simulink model "control_system"  (R2023b)
settings: Solver=VariableStepAuto  StartTime=0.0  StopTime=10.0  MaxStep=0.01  RelTol=1e-3
undefined symbols (not defined in the file): I
libraries: slpidlib x2, simulink_extras x1
settings Model: Creator=maxaz  LastModifiedBy=maxaz

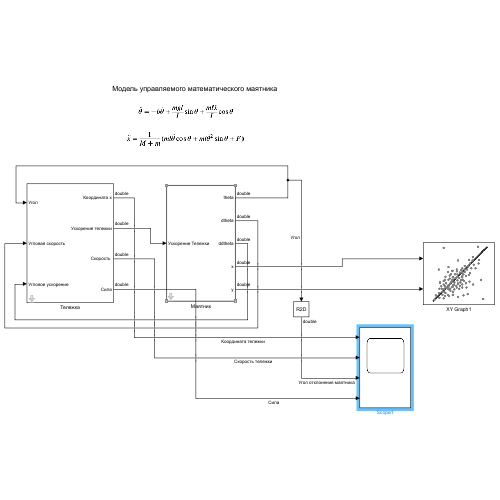
[thumbnail: Simulink's stored preview of the top-level diagram]
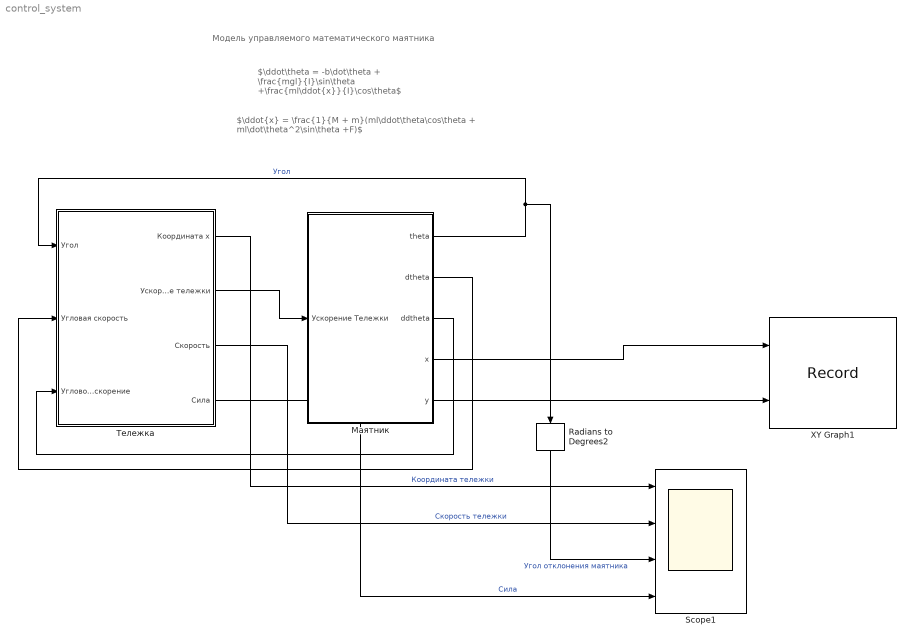
== system control_system ==
  note: Модель управляемого математического маятника
  note: $\ddot{x} = \frac{1}{M + m}(ml\ddot\theta\cos\theta + ml\dot\theta^2\sin\theta +F)$
  note: $\ddot\theta = -b\dot\theta + \frac{mgl}{I}\sin\theta +\frac{ml\ddot{x}}{I}\cos\theta$
  Radians to Degrees2 : simulink_extras/Transformations/Radians to Degrees
  Scope1 : Scope  NumInputPorts=4
  XY Graph1 : Record  FileSettingsInternal="{\"entries\":[{\"content\":{\"excelSettings\":{\"content\":{},\"type\":\"Streamout.ExcelSettings\"}},\"type\":\"Streamout.FileSettingStorage\",\"uuid\":\"\"}],\"packageUris\":[\"http:\\/\\/schema.mathworks.com\\/mf0\\/streamout_blocks\\/R2020a\"],\"version\":\"1.0\"}"  Layout=[1 1]  SignalsInternal="{\"entries\":[{\"content\":{\"signals\":[{\"content\":{\"blockPath\":[],\"dimensions\":[1],\"domain\":\"\",\"lineColor\":\"#a2142f\",\"plots\":[1],\"port\":1,\"sid\":[\"\"],\"signalID\":6168,\"signalName\":\"Маятник:4\"},\"type\":\"RecordBlkView.Signal\",\"uuid\":\"\"},{\"content\":{\"blockPath\":[],\"dimensions\":[1],\"domain\":\"\",\"lineColor\":\"#139fff\",\"plots\":[1],\"port\":2,\"sid\":[\"\"],\"signalID\":6172,\"signalName\":\"Маятник:5\"},\"type\":\"RecordBlkView.Signal\",\"uuid\":\"\"}]},\"type\":\"RecordBlkView.InputSignals\",\"uuid\":\"\"}],\"packageUris\":[\"http:\\/\\/schema.mathworks.com\\/mf0\\/streamout_blocks\\/R2020a\"],\"version\":\"1.0\"}"  VisualizationBindings="{\"xyplotplugin\":{\"info\":[{\"series\":[{\"bindingParametersList\":[{\"parameter\":\"X-Axis\",\"signalID\":6168,\"signalName\":\"Маятник:4\"},{\"parameter\":\"Y-Axis\",\"signalID\":6172,\"signalName\":\"Маятник:5\"}],\"seriesID\":9989}],\"subplotID\":1}]}}"  CompatibilityTag=XY
  Маятник : Subsystem  mask{m=1, g=9.8, l=1, startDegree=30, b=0.3}
      mask prompts: m "Масса, кг"; g "Ускорение свободного падения, м/с^2"; l "Длина, м"; startDegree "Начальный угол, градусы"; b "Диссипативный коэффициент"
  Тележка : Subsystem  mask{m=1, M_T=10, l=1, P=11, I=0, D=5.5}
      mask prompts: m "Масса маятника"; M_T "Масса тележки"; l "Длина маятника"
  wires:
  Тележка/4(Сила) -> Scope1/4  "Сила"
  Radians to Degrees2/1 -> Scope1/3  "Угол отклонения маятника"
  Тележка/3("Скорость ") -> Scope1/2  "Скорость тележки"
  Тележка/2(Ускорение тележки) -> Маятник/1(Ускорение Тележки)
  Маятник/3(ddtheta) -> Тележка/3(Угловое ускорение)
  Тележка/1(Координата x) -> Scope1/1  "Координата тележки"
  Маятник/2(dtheta) -> Тележка/2(Угловая скорость)
  Маятник/4(x) -> XY Graph1/1
  Маятник/5(y) -> XY Graph1/2
  Маятник/1(theta) -> Тележка/1(Угол), Radians to Degrees2/1  "Угол"

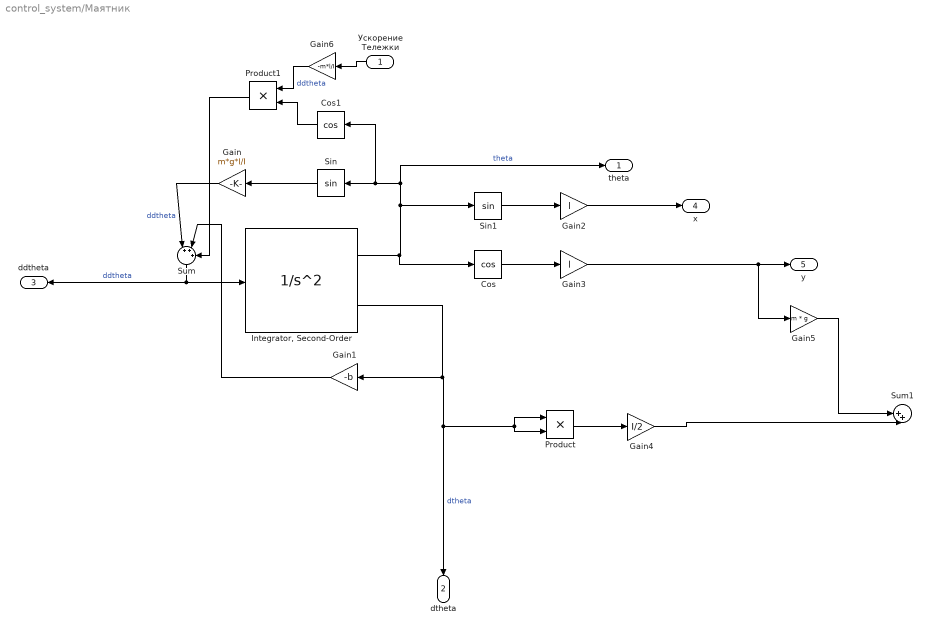
== system control_system/Маятник ==
  Ускорение Тележки : Inport
  Cos : Trigonometry  Operator=cos
  Cos1 : Trigonometry  Operator=cos
  Gain : Gain  Gain=m*g*l/I
  Gain1 : Gain  Gain=-b
  Gain2 : Gain  Gain=l
  Gain3 : Gain  Gain=l
  Gain4 : Gain  Gain=I/2
  Gain5 : Gain  Gain=m * g
  Gain6 : Gain  Gain=-m*l/I
  "Integrator, Second-Order" : SecondOrderIntegrator  ICX=deg2rad(startDegree)
  Product : Product
  Product1 : Product
  Sin : Trigonometry
  Sin1 : Trigonometry
  Sum : Sum  Inputs=|+++
  Sum1 : Sum  Inputs=|++
  theta : Outport
  dtheta : Outport  Port=2
  ddtheta : Outport  Port=3
  x : Outport  Port=4
  y : Outport  Port=5
  wires:
  "Integrator, Second-Order"/1 -> Cos/1, theta/1, Cos1/1, Sin/1, Sin1/1  "theta"
  Sin/1 -> Gain/1
  Sum/1 -> "Integrator, Second-Order"/1, ddtheta/1  "ddtheta"
  "Integrator, Second-Order"/2 -> Product/2, Product/1, dtheta/1, Gain1/1  "dtheta"
  Gain1/1 -> Sum/2
  Gain/1 -> Sum/1  "ddtheta"
  Cos/1 -> Gain3/1
  Gain2/1 -> x/1
  Sin1/1 -> Gain2/1
  Product/1 -> Gain4/1
  Gain5/1 -> Sum1/1
  Gain4/1 -> Sum1/2
  Gain3/1 -> Gain5/1, y/1
  Ускорение Тележки/1 -> Gain6/1
  Cos1/1 -> Product1/2
  Gain6/1 -> Product1/1  "ddtheta"
  Product1/1 -> Sum/3

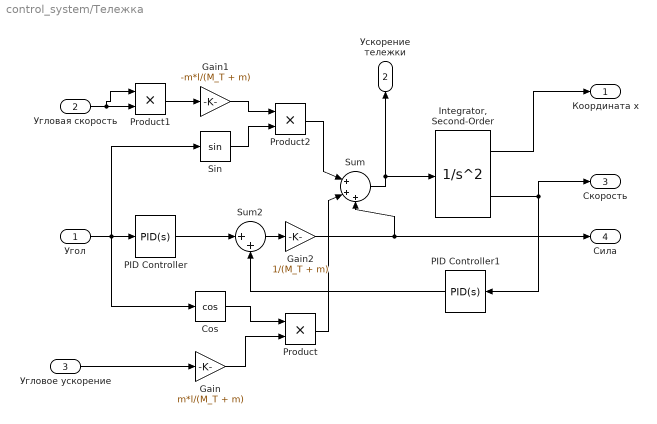
== system control_system/Тележка ==
  Угол : Inport
  Угловая скорость : Inport  Port=2
  Угловое ускорение : Inport  Port=3
  Cos : Trigonometry  Operator=cos
  Gain : Gain  Gain=m*l/(M_T + m)
  Gain1 : Gain  Gain=-m*l/(M_T + m)
  Gain2 : Gain  Gain=1/(M_T + m)
  "Integrator, Second-Order" : SecondOrderIntegrator
  PID Controller : slpidlib/PID Controller  Controller=PID  Form=Parallel  TimeDomain=Continuous-time  UseExternalTs=off  SampleTime=-1  IntegratorMethod=Forward Euler  FilterMethod=Forward Euler  ControllerParametersSource=internal  P=200  I=0  UseKiTs=off  D=50  N=100  UseFilter=on  TunerSelectOption=Transfer Function Based (PID Tuner App)  InitialConditionSource=internal  InitialConditionForIntegrator=0  InitialConditionForFilter=0  DifferentiatorICPrevScaledInput=0  ExternalReset=none  TrackingMode=off  Kt=1  LimitOutput=off  SatLimitsSource=internal  UpperSaturationLimit=inf  LowerSaturationLimit=-inf  LinearizeAsGain=on  AntiWindupMode=none  Kb=1  LimitIntegrator=off  UpperIntegratorSaturationLimit=inf  LowerIntegratorSaturationLimit=-inf  POutMin=[]  POutMax=[]  IOutMin=[]  IOutMax=[]  DOutMin=[]  DOutMax=[]  NOutMin=[]  NOutMax=[]  SumOutMin=[]  SumOutMax=[]  SaturationOutMin=[]  SaturationOutMax=[]  PParamMin=[]  PParamMax=[]  IParamMin=[]  IParamMax=[]  DParamMin=[]  DParamMax=[]  NParamMin=[]  NParamMax=[]  KbParamMin=[]  KbParamMax=[]  KtParamMin=[]  KtParamMax=[]  KbOutMin=[]  KbOutMax=[]  KtOutMin=[]  KtOutMax=[]  IntegratorOutMin=[]  IntegratorOutMax=[]  FilterOutMin=[]  FilterOutMax=[]  SumI1OutMin=[]  SumI1OutMax=[]  SumI2OutMin=[]  SumI2OutMax=[]  SumI3OutMin=[]  SumI3OutMax=[]  SumI4OutMin=[]  SumI4OutMax=[]  SumDOutMin=[]  SumDOutMax=[]  DifferentiatorOutMin=[]  DifferentiatorOutMax=[]  FilterDiffOutCoefMin=[]  FilterDiffOutCoefMax=[]  ReciprocalOutMin=[]  ReciprocalOutMax=[]  SumDenOutMin=[]  SumDenOutMax=[]  SumNumOutMin=[]  SumNumOutMax=[]  DivideOutMin=[]  DivideOutMax=[]  UdiffTsProdOutMin=[]  UdiffTsProdOutMax=[]  NTsProdOutMin=[]  NTsProdOutMax=[]  UintegralTsProdOutMin=[]  UintegralTsProdOutMax=[]  UngainTsProdOutMin=[]  UngainTsProdOutMax=[]  ClampingZeroOutDataTypeStr=Inherit: Inherit via back propagation  ClampingZeroOutMin=[]  ClampingZeroOutMax=[]  FilterDenConstantOutDataTypeStr=Inherit: Inherit via back propagation  FilterDenConstantOutMin=[]  FilterDenConstantOutMax=[]  PCopyOutDataTypeStr=Inherit: Inherit via back propagation  PCopyOutMin=[]  PCopyOutMax=[]  NCopyOutDataTypeStr=Inherit: Inherit via back propagation  NCopyOutMin=[]  NCopyOutMax=[]  IntegratorContinuousStateAttributes=''  IntegratorStateMustResolveToSignalObject=off  IntegratorRTWStateStorageClass=Auto  FilterContinuousStateAttributes=''  FilterStateMustResolveToSignalObject=off  FilterRTWStateStorageClass=Auto  ParallelPVariant=InternalParameters  IdealPVariant=Disabled  IVariant=InternalParameters  DVariant=InternalParameters  IntegratorVariant=Continuous  SatVariant=Disabled  AWVariant=Passthrough  PCopyVariant=Disabled  TRVariant=Disabled  FdbkBlocksVariant=Forward  IdealPFdbkVariant=Disabled  SatFdbkVariant=Disabled  DerivativeFilterVariant=ContFilter  NVariant=InternalParameters  NCopyVariant=Disabled  FilterICVariant=InternalICsFilter  IntegratorICVariant=InternalICs  ExternalResetVariant=Disabled  TRSumVariant=Passthrough  SumFdbkVariant=Disabled  SumVariant=Sum_PID  TsampFilterVariant=InternalTs  TsampNgainVariant=Passthrough  TsampIntegralVariant=Disabled_SignalSpec  ExternalSaturationOutDataTypeStr=Inherit: Same as second input
  PID Controller1 : slpidlib/PID Controller  Controller=PID  Form=Parallel  TimeDomain=Continuous-time  UseExternalTs=off  SampleTime=-1  IntegratorMethod=Forward Euler  FilterMethod=Forward Euler  ControllerParametersSource=internal  P=P  I=I  UseKiTs=off  D=D  N=100  UseFilter=on  TunerSelectOption=Transfer Function Based (PID Tuner App)  InitialConditionSource=internal  InitialConditionForIntegrator=0  InitialConditionForFilter=0  DifferentiatorICPrevScaledInput=0  ExternalReset=none  TrackingMode=off  Kt=1  LimitOutput=off  SatLimitsSource=internal  UpperSaturationLimit=inf  LowerSaturationLimit=-inf  LinearizeAsGain=on  AntiWindupMode=none  Kb=1  LimitIntegrator=off  UpperIntegratorSaturationLimit=inf  LowerIntegratorSaturationLimit=-inf  POutMin=[]  POutMax=[]  IOutMin=[]  IOutMax=[]  DOutMin=[]  DOutMax=[]  NOutMin=[]  NOutMax=[]  SumOutMin=[]  SumOutMax=[]  SaturationOutMin=[]  SaturationOutMax=[]  PParamMin=[]  PParamMax=[]  IParamMin=[]  IParamMax=[]  DParamMin=[]  DParamMax=[]  NParamMin=[]  NParamMax=[]  KbParamMin=[]  KbParamMax=[]  KtParamMin=[]  KtParamMax=[]  KbOutMin=[]  KbOutMax=[]  KtOutMin=[]  KtOutMax=[]  IntegratorOutMin=[]  IntegratorOutMax=[]  FilterOutMin=[]  FilterOutMax=[]  SumI1OutMin=[]  SumI1OutMax=[]  SumI2OutMin=[]  SumI2OutMax=[]  SumI3OutMin=[]  SumI3OutMax=[]  SumI4OutMin=[]  SumI4OutMax=[]  SumDOutMin=[]  SumDOutMax=[]  DifferentiatorOutMin=[]  DifferentiatorOutMax=[]  FilterDiffOutCoefMin=[]  FilterDiffOutCoefMax=[]  ReciprocalOutMin=[]  ReciprocalOutMax=[]  SumDenOutMin=[]  SumDenOutMax=[]  SumNumOutMin=[]  SumNumOutMax=[]  DivideOutMin=[]  DivideOutMax=[]  UdiffTsProdOutMin=[]  UdiffTsProdOutMax=[]  NTsProdOutMin=[]  NTsProdOutMax=[]  UintegralTsProdOutMin=[]  UintegralTsProdOutMax=[]  UngainTsProdOutMin=[]  UngainTsProdOutMax=[]  ClampingZeroOutDataTypeStr=Inherit: Inherit via back propagation  ClampingZeroOutMin=[]  ClampingZeroOutMax=[]  FilterDenConstantOutDataTypeStr=Inherit: Inherit via back propagation  FilterDenConstantOutMin=[]  FilterDenConstantOutMax=[]  PCopyOutDataTypeStr=Inherit: Inherit via back propagation  PCopyOutMin=[]  PCopyOutMax=[]  NCopyOutDataTypeStr=Inherit: Inherit via back propagation  NCopyOutMin=[]  NCopyOutMax=[]  IntegratorContinuousStateAttributes=''  IntegratorStateMustResolveToSignalObject=off  IntegratorRTWStateStorageClass=Auto  FilterContinuousStateAttributes=''  FilterStateMustResolveToSignalObject=off  FilterRTWStateStorageClass=Auto  ParallelPVariant=InternalParameters  IdealPVariant=Disabled  IVariant=InternalParameters  DVariant=InternalParameters  IntegratorVariant=Continuous  SatVariant=Disabled  AWVariant=Passthrough  PCopyVariant=Disabled  TRVariant=Disabled  FdbkBlocksVariant=Forward  IdealPFdbkVariant=Disabled  SatFdbkVariant=Disabled  DerivativeFilterVariant=ContFilter  NVariant=InternalParameters  NCopyVariant=Disabled  FilterICVariant=InternalICsFilter  IntegratorICVariant=InternalICs  ExternalResetVariant=Disabled  TRSumVariant=Passthrough  SumFdbkVariant=Disabled  SumVariant=Sum_PID  TsampFilterVariant=InternalTs  TsampNgainVariant=Passthrough  TsampIntegralVariant=Disabled_SignalSpec  ExternalSaturationOutDataTypeStr=Inherit: Same as second input
  Product : Product
  Product1 : Product
  Product2 : Product
  Sin : Trigonometry
  Sum : Sum  Inputs=|+++
  Sum2 : Sum  Inputs=|++
  Координата x : Outport
  Ускорение тележки : Outport  Port=2
  "Скорость " : Outport  Port=3
  Сила : Outport  Port=4
  wires:
  Угловое ускорение/1 -> Gain/1
  "Integrator, Second-Order"/1 -> Координата x/1
  Угловая скорость/1 -> Product1/1, Product1/2
  Угол/1 -> Cos/1, Sin/1, PID Controller/1
  Gain/1 -> Product/2
  Cos/1 -> Product/1
  Product1/1 -> Gain1/1
  Sin/1 -> Product2/2
  Gain1/1 -> Product2/1
  Product/1 -> Sum/2
  Product2/1 -> Sum/1
  Sum/1 -> Ускорение тележки/1, "Integrator, Second-Order"/1
  "Integrator, Second-Order"/2 -> "Скорость "/1, PID Controller1/1
  PID Controller1/1 -> Sum2/2
  Sum2/1 -> Gain2/1
  Gain2/1 -> Sum/3, Сила/1
  PID Controller/1 -> Sum2/1
